simulink model "test_liniearization"  (R2024b)
settings: Solver=VariableStepAuto  StartTime=0.0  StopTime=500  RelTol=1e-3
values from neighbouring files (symbols this model uses):
  theta0 = 0.0604    [RCAM_get_linearmodel_from_optrim_HS.m]
  u0 = V*cos(alpha)    [RCAM_get_linearmodel_from_optrim_HS.m]
undefined symbols (not defined in the file or in its folder): A_new, alpha0, B_new, C_lon, D_lon, q0, RCAM_dynamics_fcn
settings Model: Creator=rukky  LastModifiedBy=kiriki

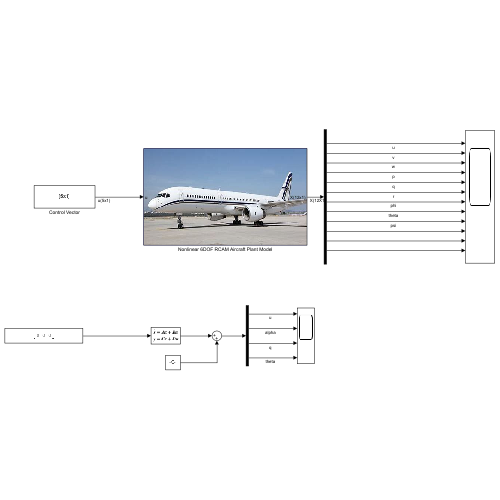
[thumbnail: Simulink's stored preview of the top-level diagram]
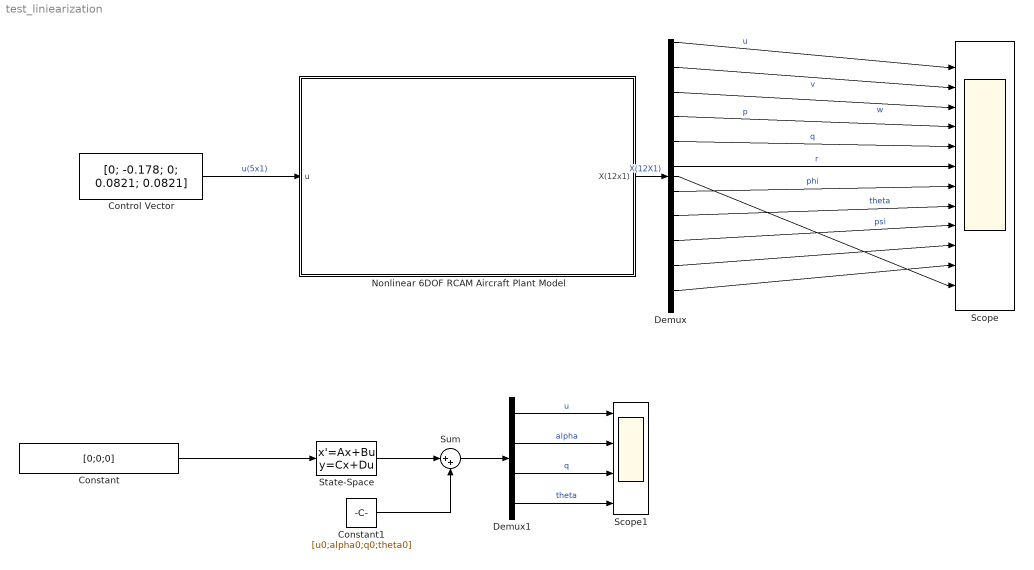
== system test_liniearization ==
  Constant : Constant  Value=[0;0;0]
  Constant1 : Constant  Value=[u0;alpha0;q0;theta0]
  Control Vector : Constant  Value=[0; -0.178; 0; 0.0821; 0.0821]
  Demux : Demux  Outputs=12
  Demux1 : Demux
  Nonlinear 6DOF RCAM Aircraft Plant Model : Subsystem
      mask Display: image('$imagefile'); % Use "Edit Image" on toolstrip to change.
  Scope : Scope  NumInputPorts=12
  Scope1 : Scope  NumInputPorts=4
  State-Space : StateSpace  A=A_new  B=B_new  C=C_lon  D=D_lon  InitialCondition=0
  Sum : Sum  Inputs=|++
  wires:
  Nonlinear 6DOF RCAM Aircraft Plant Model/1(X(12x1)) -> Demux/1  "X(12X1)"
  Control Vector/1 -> Nonlinear 6DOF RCAM Aircraft Plant Model/1(u)  "u(5x1)"
  Demux/1 -> Scope/1  "u"
  Demux/2 -> Scope/2  "v"
  Demux/3 -> Scope/3  "w"
  Demux/4 -> Scope/4  "p"
  Demux/5 -> Scope/5  "q"
  Demux/6 -> Scope/6  "r"
  Demux/7 -> Scope/7  "phi"
  Demux/8 -> Scope/8  "theta"
  Demux/9 -> Scope/9  "psi"
  Demux/10 -> Scope/10
  Demux/11 -> Scope/11
  Demux/12 -> Scope/12
  Constant/1 -> State-Space/1
  State-Space/1 -> Sum/1
  Demux1/4 -> Scope1/4  "theta"
  Demux1/1 -> Scope1/1  "u"
  Demux1/2 -> Scope1/2  "alpha"
  Demux1/3 -> Scope1/3  "q"
  Sum/1 -> Demux1/1
  Constant1/1 -> Sum/2

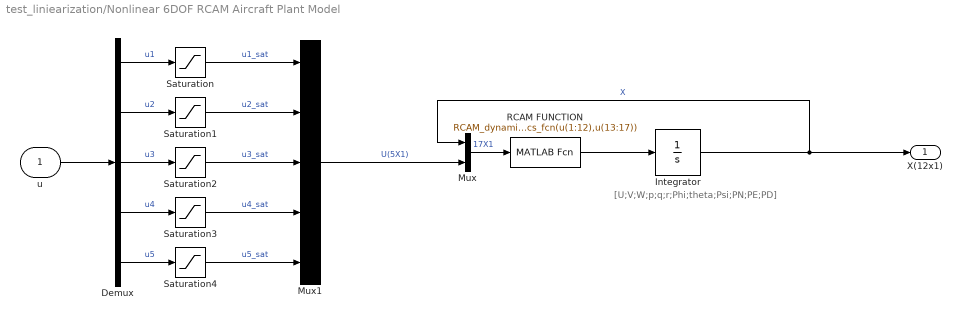
== system test_liniearization/Nonlinear 6DOF RCAM Aircraft Plant Model ==
  note: [U;V;W;p;q;r;Phi;theta;Psi;PN;PE;PD]
  u : Inport
  Demux : Demux  Outputs=5
  Integrator : Integrator  InitialCondition=|
      | [84.9905; 0;
      |  1.2713;
      | 0; 0; 0; 0; 0.1; 0; 0; 0.0149; 0]
  Mux : Mux  Inputs=2
  Mux1 : Mux  Inputs=5
  RCAM FUNCTION : MATLABFcn  MATLABFcn=RCAM_dynamics_fcn(u(1:12),u(13:17))
  Saturation : Saturate  UpperLimit=25*(pi/180)  LowerLimit=-15*(pi/180)
  Saturation1 : Saturate  UpperLimit=10*(pi/180)  LowerLimit=-25*(pi/180)
  Saturation2 : Saturate  UpperLimit=30*(pi/180)  LowerLimit=-30*(pi/180)
  Saturation3 : Saturate  UpperLimit=10*(pi/180)  LowerLimit=0.5*(pi/180)
  Saturation4 : Saturate  UpperLimit=10*(pi/180)  LowerLimit=0.5*(pi/180)
  X(12x1) : Outport
  wires:
  Integrator/1 -> Mux/1, X(12x1)/1  "X"
  u/1 -> Demux/1
  Demux/1 -> Saturation/1  "u1"
  Saturation/1 -> Mux1/1  "u1_sat"
  Demux/2 -> Saturation1/1  "u2"
  Demux/3 -> Saturation2/1  "u3"
  Demux/4 -> Saturation3/1  "u4"
  Demux/5 -> Saturation4/1  "u5"
  Saturation1/1 -> Mux1/2  "u2_sat"
  Saturation2/1 -> Mux1/3  "u3_sat"
  Saturation3/1 -> Mux1/4  "u4_sat"
  Saturation4/1 -> Mux1/5  "u5_sat"
  RCAM FUNCTION/1 -> Integrator/1
  Mux/1 -> RCAM FUNCTION/1  "17X1"
  Mux1/1 -> Mux/2  "U(5X1)"
